simulink model "centroid_model"  (R2022b)
settings: Solver=VariableStepAuto  StartTime=0.0  StopTime=10  RelTol=1e-3
values from neighbouring files (symbols this model uses):
  k1 = 0.4    [centroid_control.m]
  k2 = 0.8    [centroid_control.m]
  k3 = 0.1    [centroid_control.m]
  q_i_1 = [-1 -1 0]'    [centroid_control.m]
  q_i_2 = [-2 1 0]'    [centroid_control.m]
  Ts = 0.1    [centroid_control.m]
libraries: robotmobilelib x2
settings Model: Creator=gaetano  LastModifiedBy=gaetano

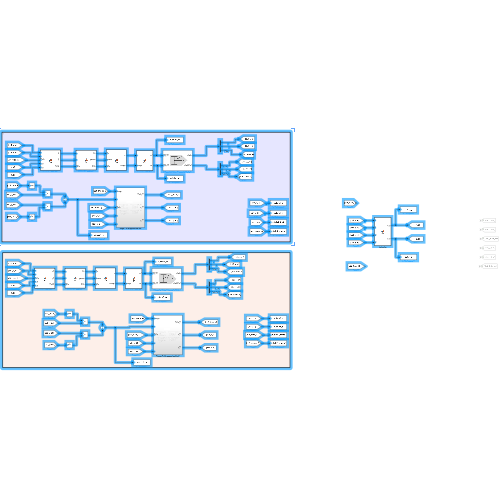
[thumbnail: Simulink's stored preview of the top-level diagram]
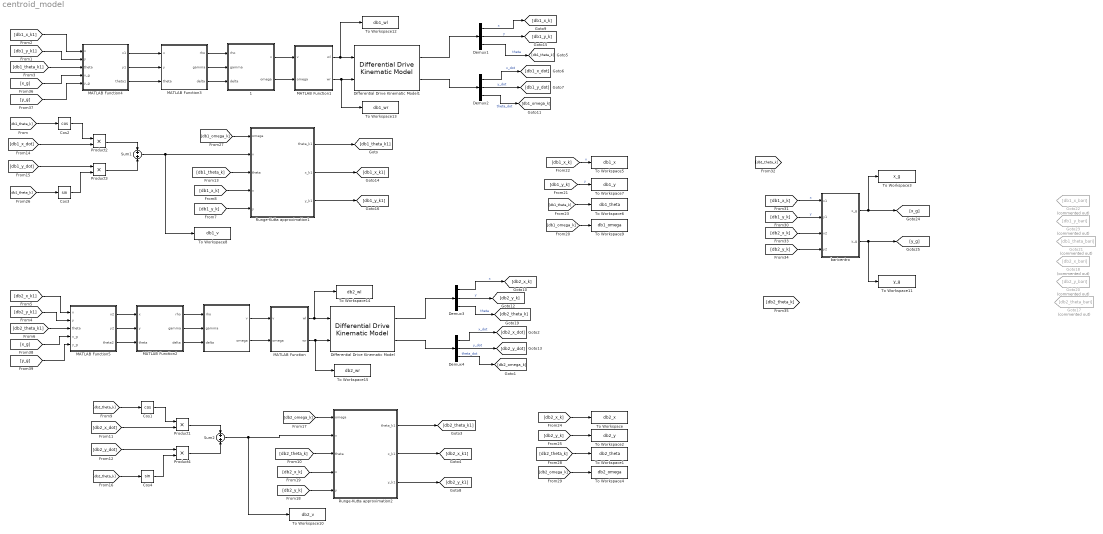
== system centroid_model ==
  " " : MATLAB Function  TreatAsAtomicUnit=on
  " 1" : MATLAB Function  TreatAsAtomicUnit=on
  Cos1 : Trigonometry  Operator=cos
  Cos2 : Trigonometry  Operator=cos
  Cos3 : Trigonometry
  Cos4 : Trigonometry
  Demux{1..4} (4 alike) : Demux  Outputs=3
  Differential Drive Kinematic Model : robotmobilelib/Differential Drive Kinematic Model  VehicleInputs=Wheel Speeds  WheelRadius=0.0318  WheelSpeedRange=[-inf inf]  TrackWidth=0.1232  InitialState=q_i_2  SimulateUsing=Interpreted execution
  Differential Drive Kinematic Model1 : robotmobilelib/Differential Drive Kinematic Model  VehicleInputs=Wheel Speeds  WheelRadius=0.0318  WheelSpeedRange=[-inf inf]  TrackWidth=0.1232  InitialState=q_i_1  SimulateUsing=Interpreted execution
  Goto17 : Goto  Commented=on  GotoTag=db2_theta_bari
  Goto18 : Goto  Commented=on  GotoTag=db2_x_bari
  Goto20 : Goto  Commented=on  GotoTag=db2_y_bari
  Goto21 : Goto  Commented=on  GotoTag=db1_theta_bari
  Goto22 : Goto  Commented=on  GotoTag=db1_x_bari
  Goto23 : Goto  Commented=on  GotoTag=db1_y_bari
  MATLAB Function : MATLAB Function  TreatAsAtomicUnit=on
  MATLAB Function1 : MATLAB Function  TreatAsAtomicUnit=on
  MATLAB Function2 : MATLAB Function  TreatAsAtomicUnit=on
  MATLAB Function3 : MATLAB Function  TreatAsAtomicUnit=on
  MATLAB Function4 : MATLAB Function  TreatAsAtomicUnit=on
  MATLAB Function5 : MATLAB Function  TreatAsAtomicUnit=on
  Product{1..4} (4 alike) : Product
  Runge-Kutta approximation1 : Subsystem
  Runge-Kutta approximation2 : Subsystem
  Sum1 : Sum  Inputs=+|+
  Sum2 : Sum  Inputs=+|+
  To Workspace : ToWorkspace  VariableName=db2_x  SaveFormat=Timeseries  SampleTime=-1
  To Workspace1 : ToWorkspace  VariableName=db2_theta  SaveFormat=Timeseries  SampleTime=-1
  To Workspace10 : ToWorkspace  VariableName=db2_v  SaveFormat=Timeseries  SampleTime=-1
  To Workspace11 : ToWorkspace  VariableName=y_g  SaveFormat=Timeseries  SampleTime=-1
  To Workspace12 : ToWorkspace  VariableName=db1_wl  SaveFormat=Timeseries  SampleTime=-1
  To Workspace13 : ToWorkspace  VariableName=db1_wr  SaveFormat=Timeseries  SampleTime=-1
  To Workspace14 : ToWorkspace  VariableName=db2_wl  SaveFormat=Timeseries  SampleTime=-1
  To Workspace15 : ToWorkspace  VariableName=db2_wr  SaveFormat=Timeseries  SampleTime=-1
  To Workspace2 : ToWorkspace  VariableName=db2_y  SaveFormat=Timeseries  SampleTime=-1
  To Workspace3 : ToWorkspace  VariableName=x_g  SaveFormat=Timeseries  SampleTime=-1
  To Workspace4 : ToWorkspace  VariableName=db2_omega  SaveFormat=Timeseries  SampleTime=-1
  To Workspace5 : ToWorkspace  VariableName=db1_x  SaveFormat=Timeseries  SampleTime=-1
  To Workspace6 : ToWorkspace  VariableName=db1_theta  SaveFormat=Timeseries  SampleTime=-1
  To Workspace7 : ToWorkspace  VariableName=db1_y  SaveFormat=Timeseries  SampleTime=-1
  To Workspace8 : ToWorkspace  VariableName=db1_v  SaveFormat=Timeseries  SampleTime=-1
  To Workspace9 : ToWorkspace  VariableName=db1_omega  SaveFormat=Timeseries  SampleTime=-1
  baricentro : MATLAB Function  TreatAsAtomicUnit=on
  wires:
  " "/2(omega) -> MATLAB Function/2(omega)
  " "/1(v) -> MATLAB Function/1(v)
  MATLAB Function2/2(gamma) -> " "/2(gamma)
  MATLAB Function2/3(delta) -> " "/3(delta)
  MATLAB Function2/1(rho) -> " "/1(rho)
  MATLAB Function/1(wl) -> To Workspace14/1, Differential Drive Kinematic Model/1
  MATLAB Function/2(wr) -> To Workspace15/1, Differential Drive Kinematic Model/2
  Demux3/2 -> [db2_y_k]  "y"
  Demux4/1 -> [db2_x_dot]  "x_dot"
  Differential Drive Kinematic Model/2 -> Demux4/1
  Differential Drive Kinematic Model/1 -> Demux3/1
  Demux3/3 -> [db2_theta_k]  "theta"
  Demux4/3 -> [db2_omega_k]  "theta_dot"
  Demux3/1 -> [db2_x_k]  "x"
  Demux4/2 -> [db2_y_dot]  "y_dot"
  MATLAB Function3/1(rho) -> " 1"/1(rho)
  Differential Drive Kinematic Model1/1 -> Demux1/1
  Differential Drive Kinematic Model1/2 -> Demux2/1
  Demux2/2 -> [db1_y_dot]  "y_dot"
  MATLAB Function3/3(delta) -> " 1"/3(delta)
  MATLAB Function4/1(x1) -> MATLAB Function3/1(x)
  MATLAB Function3/2(gamma) -> " 1"/2(gamma)
  " 1"/1(v) -> MATLAB Function1/1(v)
  MATLAB Function1/1(wl) -> To Workspace12/1, Differential Drive Kinematic Model1/1
  MATLAB Function4/2(y1) -> MATLAB Function3/2(y)
  MATLAB Function1/2(wr) -> To Workspace13/1, Differential Drive Kinematic Model1/2
  " 1"/2(omega) -> MATLAB Function1/2(omega)
  Demux1/1 -> [db1_x_k]  "x"
  Demux2/1 -> [db1_x_dot]  "x_dot"
  MATLAB Function4/3(theta1) -> MATLAB Function3/3(theta)
  Demux2/3 -> [db1_omega_k]  "theta_dot"
  Demux1/2 -> [db1_y_k]  "y"
  Runge-Kutta approximation1/1(theta_k1) -> [db1_theta_k1]
  [db1_x_k] -> Runge-Kutta approximation1/4(x)
  [db1_theta_k] -> Runge-Kutta approximation1/3(theta)
  Cos2/1 -> Product2/1
  Product3/1 -> Sum1/2
  [db1_x_dot] -> Product2/2
  [db1_theta_k] -> Cos2/1
  Product2/1 -> Sum1/1
  Runge-Kutta approximation1/2(x_k1) -> [db1_x_k1]
  [db1_y_k] -> Runge-Kutta approximation1/5(y)
  [db1_omega_k] -> Runge-Kutta approximation1/1(omega)
  [db1_theta_k] -> Cos3/1
  Sum1/1 -> To Workspace8/1, Runge-Kutta approximation1/2(v)
  Cos3/1 -> Product3/2
  [db1_y_dot] -> Product3/1
  Demux1/3 -> [db1_theta_k]  "theta"
  Runge-Kutta approximation1/3(y_k1) -> [db1_y_k1]
  Runge-Kutta approximation2/3(y_k1) -> [db2_y_k1]
  [db2_theta_k] -> Runge-Kutta approximation2/3(theta)
  [db2_x_dot] -> Product1/2
  Sum2/1 -> To Workspace10/1, Runge-Kutta approximation2/2(v)
  Cos1/1 -> Product1/1
  [db2_x_k] -> Runge-Kutta approximation2/4(x)
  Product1/1 -> Sum2/1
  Product4/1 -> Sum2/2
  [db2_theta_k] -> Cos1/1
  Cos4/1 -> Product4/2
  [db2_y_k] -> Runge-Kutta approximation2/5(y)
  [db2_y_dot] -> Product4/1
  [db2_omega_k] -> Runge-Kutta approximation2/1(omega)
  [db2_theta_k] -> Cos4/1
  Runge-Kutta approximation2/1(theta_k1) -> [db2_theta_k1]
  Runge-Kutta approximation2/2(x_k1) -> [db2_x_k1]
  [db1_y_k] -> To Workspace7/1  "y"
  [db1_x_k] -> To Workspace5/1  "x"
  [db1_theta_k] -> To Workspace6/1
  [db2_x_k] -> To Workspace/1
  [db2_theta_k] -> To Workspace1/1
  [db2_y_k] -> To Workspace2/1
  [db2_omega_k] -> To Workspace4/1
  [db1_x_k] -> baricentro/1(x1)  "x"
  [db1_y_k] -> baricentro/2(y1)  "y"
  [db2_x_k] -> baricentro/3(x2)
  [db2_y_k] -> baricentro/4(y2)
  baricentro/1(x_g) -> [x_g], To Workspace3/1
  baricentro/2(y_g) -> [y_g], To Workspace11/1
  [db1_omega_k] -> To Workspace9/1
  [db1_x_k1] -> MATLAB Function4/1(x)
  [db1_y_k1] -> MATLAB Function4/2(y)
  [db1_theta_k1] -> MATLAB Function4/3(theta)
  [x_g] -> MATLAB Function4/4(x_g)
  [y_g] -> MATLAB Function4/5(y_g)
  [x_g] -> MATLAB Function5/4(x_g)
  [y_g] -> MATLAB Function5/5(y_g)
  MATLAB Function5/1(x2) -> MATLAB Function2/1(x)
  MATLAB Function5/2(y2) -> MATLAB Function2/2(y)
  MATLAB Function5/3(theta2) -> MATLAB Function2/3(theta)
  [db2_x_k1] -> MATLAB Function5/1(x)
  [db2_theta_k1] -> MATLAB Function5/3(theta)
  [db2_y_k1] -> MATLAB Function5/2(y)

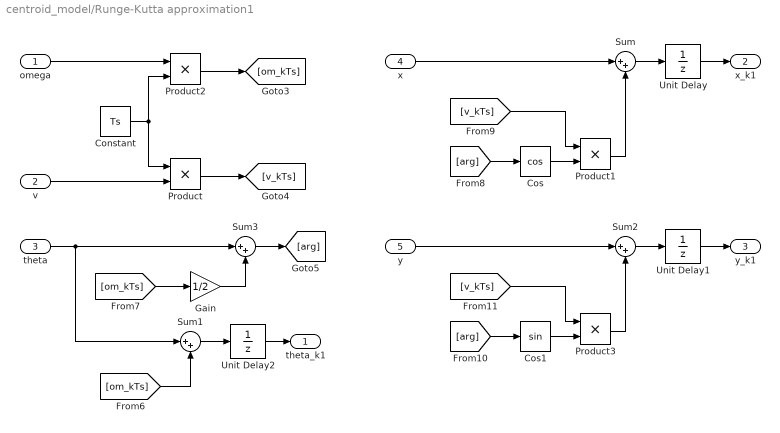
== system centroid_model/Runge-Kutta approximation1 ==
  omega : Inport
  v : Inport  Port=2
  theta : Inport  Port=3
  x : Inport  Port=4
  y : Inport  Port=5
  Constant : Constant  Value=Ts
  Cos : Trigonometry  Operator=cos
  Cos1 : Trigonometry
  Gain : Gain  Gain=1/2
  Product{,1..3} (4 alike) : Product
  Sum{,1..3} (4 alike) : Sum  Inputs=|++
  Unit Delay : UnitDelay  InitialCondition=q_i_1(1)  SampleTime=Ts  HasFrameUpgradeWarning=on
  Unit Delay1 : UnitDelay  InitialCondition=q_i_1(2)  SampleTime=Ts  HasFrameUpgradeWarning=on
  Unit Delay2 : UnitDelay  InitialCondition=q_i_1(3)  SampleTime=Ts  HasFrameUpgradeWarning=on
  theta_k1 : Outport
  x_k1 : Outport  Port=2
  y_k1 : Outport  Port=3
  wires:
  Sum3/1 -> [arg]
  theta/1 -> Sum1/1, Sum3/1
  [v_kTs] -> Product3/1
  omega/1 -> Product2/1
  [om_kTs] -> Sum1/2
  [arg] -> Cos1/1
  [arg] -> Cos/1
  x/1 -> Sum/1
  Product/1 -> [v_kTs]
  y/1 -> Sum2/1
  [om_kTs] -> Gain/1
  v/1 -> Product/2
  [v_kTs] -> Product1/1
  Cos/1 -> Product1/2
  Constant/1 -> Product2/2, Product/1
  Product2/1 -> [om_kTs]
  Product1/1 -> Sum/2
  Product3/1 -> Sum2/2
  Gain/1 -> Sum3/2
  Cos1/1 -> Product3/2
  Sum1/1 -> Unit Delay2/1
  Sum2/1 -> Unit Delay1/1
  Sum/1 -> Unit Delay/1
  Unit Delay2/1 -> theta_k1/1
  Unit Delay/1 -> x_k1/1
  Unit Delay1/1 -> y_k1/1

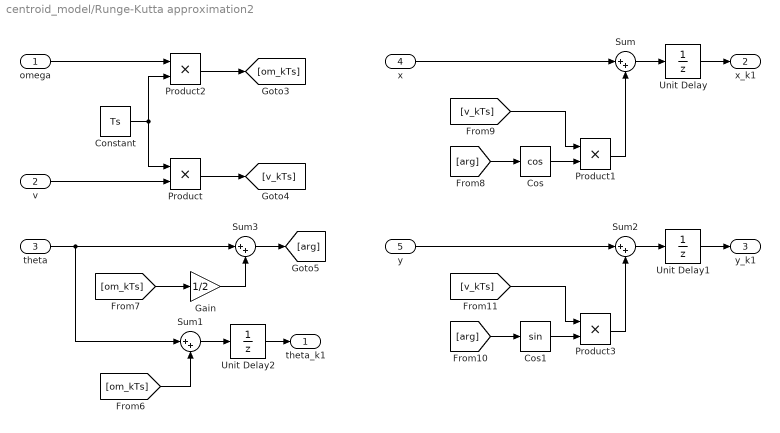
== system centroid_model/Runge-Kutta approximation2 ==
  omega : Inport
  v : Inport  Port=2
  theta : Inport  Port=3
  x : Inport  Port=4
  y : Inport  Port=5
  Constant : Constant  Value=Ts
  Cos : Trigonometry  Operator=cos
  Cos1 : Trigonometry
  Gain : Gain  Gain=1/2
  Product{,1..3} (4 alike) : Product
  Sum{,1..3} (4 alike) : Sum  Inputs=|++
  Unit Delay : UnitDelay  InitialCondition=q_i_2(1)  SampleTime=Ts  HasFrameUpgradeWarning=on
  Unit Delay1 : UnitDelay  InitialCondition=q_i_2(2)  SampleTime=Ts  HasFrameUpgradeWarning=on
  Unit Delay2 : UnitDelay  InitialCondition=q_i_2(3)  SampleTime=Ts  HasFrameUpgradeWarning=on
  theta_k1 : Outport
  x_k1 : Outport  Port=2
  y_k1 : Outport  Port=3
  wires:
  Sum3/1 -> [arg]
  theta/1 -> Sum1/1, Sum3/1
  [v_kTs] -> Product3/1
  omega/1 -> Product2/1
  [om_kTs] -> Sum1/2
  [arg] -> Cos1/1
  [arg] -> Cos/1
  x/1 -> Sum/1
  Product/1 -> [v_kTs]
  y/1 -> Sum2/1
  [om_kTs] -> Gain/1
  v/1 -> Product/2
  [v_kTs] -> Product1/1
  Cos/1 -> Product1/2
  Constant/1 -> Product2/2, Product/1
  Product2/1 -> [om_kTs]
  Product1/1 -> Sum/2
  Product3/1 -> Sum2/2
  Gain/1 -> Sum3/2
  Cos1/1 -> Product3/2
  Sum1/1 -> Unit Delay2/1
  Sum2/1 -> Unit Delay1/1
  Sum/1 -> Unit Delay/1
  Unit Delay2/1 -> theta_k1/1
  Unit Delay/1 -> x_k1/1
  Unit Delay1/1 -> y_k1/1

== matlab function centroid_model/MATLAB Function5 ==
  data: x input; x2 output; y2 output; y input; theta input; theta2 output; x_g input; y_g input; OFFSET parameter
function [x2,y2,theta2] = fcn(x,y,theta,x_g,y_g, OFFSET)

offx = (x-x_g);
offy = (y-y_g) - OFFSET;

x2 = x + offx;
y2 = y + offy;
theta2 = theta;

== matlab function centroid_model/ 1 ==
  data: rho input; v output; omega output; gamma input; delta input; k1 parameter; k2 parameter; k3 parameter
function [v,omega] = fcn(rho,gamma,delta, k1, k2, k3)

v = k1 * rho * cos(gamma);
omega = k2 * gamma + k1*sin(gamma)*cos(gamma)*(1+k3*delta/gamma);

== matlab function centroid_model/MATLAB Function ==
  data: wl output; v input; omega input; wr output
function [wl, wr] = fcn(v, omega)

 raggio = 0.0318;
 interasse = 0.1232;

	wr = (2*v + omega*interasse)/(2*raggio);
	wl = (2*v - omega*interasse)/(2*raggio);

end

== matlab function centroid_model/MATLAB Function2 ==
  data: x input; rho output; gamma output; y input; theta input; delta output
function [rho,gamma,delta] = fcn(x,y,theta)

rho = sqrt(x^2+y^2);

gamma = atan2(y,x) - theta + pi;
% gamma = mod(gamma + pi, 2*pi) - pi;
    while gamma > pi
        gamma = gamma - 2*pi;
    end
    
    while gamma < -pi
        gamma = gamma + 2*pi;
    end

delta = gamma + theta;

== matlab function centroid_model/  ==
  data: rho input; v output; omega output; gamma input; delta input; k1 parameter; k2 parameter; k3 parameter
function [v,omega] = fcn(rho,gamma,delta, k1, k2, k3)

v = k1 * rho * cos(gamma);
omega = k2 * gamma + k1*sin(gamma)*cos(gamma)*(1+k3*delta/gamma);

== matlab function centroid_model/MATLAB Function1 ==
  data: wl output; v input; omega input; wr output
function [wl, wr] = fcn(v, omega)

 raggio = 0.0318;
 interasse = 0.1232;

	wr = (2*v + omega*interasse)/(2*raggio);
	wl = (2*v - omega*interasse)/(2*raggio);

end

== matlab function centroid_model/MATLAB Function3 ==
  data: x input; rho output; gamma output; y input; theta input; delta output
function [rho,gamma,delta] = fcn(x,y,theta)

rho = sqrt(x^2+y^2);

gamma = atan2(y,x) - theta + pi;
% gamma = mod(gamma + pi, 2*pi) - pi;
    while gamma > pi
        gamma = gamma - 2*pi;
    end
    
    while gamma < -pi
        gamma = gamma + 2*pi;
    end

delta = gamma + theta;

== matlab function centroid_model/baricentro ==
  data: x1 input; x_g output; y1 input; x2 input; y2 input; y_g output
function [x_g,y_g] = fcn(x1,y1,x2,y2)

x_g = (x1+x2)/2;
y_g = (y1+y2)/2;

== matlab function centroid_model/MATLAB Function4 ==
  data: x input; x1 output; y1 output; y input; theta input; theta1 output; x_g input; y_g input; OFFSET parameter
function [x1,y1,theta1] = fcn(x,y,theta,x_g,y_g, OFFSET)

offx = (x-x_g);
offy = (y-y_g) + OFFSET;

x1 = x + offx;
y1 = y + offy;
theta1 = theta;
